simulink model "MarsEntry2"  (R2026a)
settings: Solver=ode45  StopTime=500  MaxStep=1  RelTol=1e-9  AbsTol=1e-10
settings Model: Creator=Ashwin  LastModifiedBy=aganesh
settings SFSimCC: SimGPUStackLimitPerThread=51200.0
settings RTWCC: GPUStackLimitPerThread=51200.0

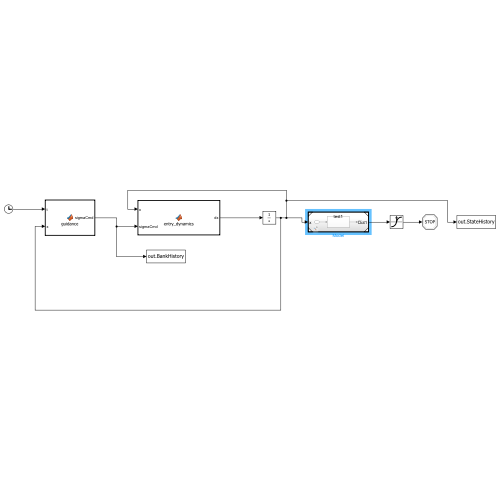
[thumbnail: Simulink's stored preview of the top-level diagram]
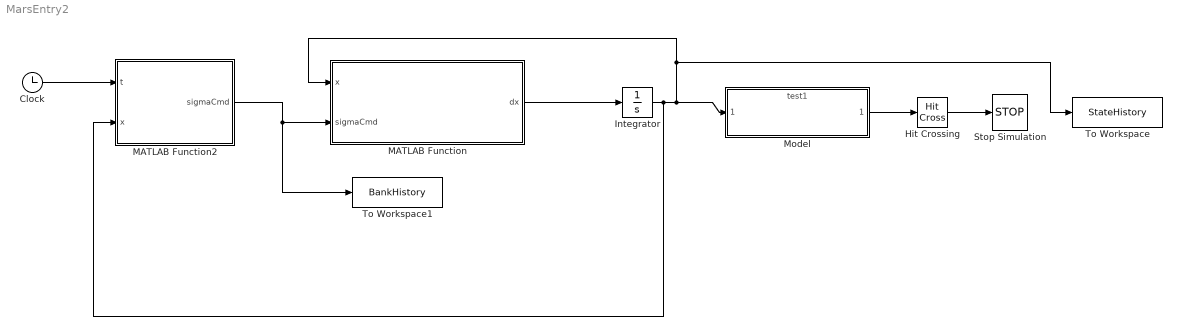
== system MarsEntry2 ==
  Clock : Clock
  Hit Crossing : HitCross  HitCrossingDirection=rising
  Integrator : Integrator  InitialCondition=[3397e3+125e3; -176.4*pi/180; -21.3*pi/180; 4700; -10*pi/180; -2.876*pi/180; 0]
  MATLAB Function : MATLAB Function  TreatAsAtomicUnit=on
  MATLAB Function2 : MATLAB Function  TreatAsAtomicUnit=on
  Model : ModelReference  ModelNameDialog=test1.slx  SimulationMode=Normal  ModelReferenceVersion=1.2
  Stop Simulation : Stop
  To Workspace : ToWorkspace  VariableName=StateHistory  SaveFormat=Timeseries  SampleTime=-1
  To Workspace1 : ToWorkspace  VariableName=BankHistory  SaveFormat=Timeseries  SampleTime=-1
  wires:
  MATLAB Function2/1(sigmaCmd) -> MATLAB Function/2(sigmaCmd), To Workspace1/1
  MATLAB Function/1(dx) -> Integrator/1
  Integrator/1 -> Model/1, MATLAB Function/1(x), To Workspace/1, MATLAB Function2/2(x)
  Clock/1 -> MATLAB Function2/1(t)
  Hit Crossing/1 -> Stop Simulation/1
  Model/1 -> Hit Crossing/1

== matlab function MarsEntry2/MATLAB Function2 ==
  settings: updateMethod=DISCRETE  sampleTime=1
  data: t input; sigmaCmd output; x input
function sigmaCmd = guidance(t,x)

coder.extrinsic('anpcg_update');
coder.extrinsic('anpcg_bank_direction');

persistent previousBank previousSign

if isempty(previousBank)
    previousBank = 100*pi/180;

    % Positive initial bank for this mission's heading error.
    previousSign = 1;
end

sigmaCmd = 0;

if t >= 175

    % Longitudinal guidance: determine bank magnitude
    nextBank = 0;
    nextBank = anpcg_update(x,previousBank);

    % Lateral guidance: determine bank direction
    nextSign = 1;
    nextSign = anpcg_bank_direction(x,nextBank,previousSign);

    previousBank = nextBank;
    previousSign = nextSign;

    sigmaCmd = nextSign*nextBank;
end

end

== matlab function MarsEntry2/MATLAB Function ==
  data: x input; dx output; sigmaCmd input
function dx = entry_dynamics(x, sigmaCmd)
% States: [r; theta; phi; V; gamma; psi; s]
% Distances in meters, time in seconds, angles in radians.

%% Mars constants
RMars = 3397e3;
mu    = 42828e9;
omega = 7.088e-5;

%% Human-mission vehicle
mass = 58800;
S    = 160;
CL   = 0.5236;
CD   = 0.9696;

beta = mass/(CD*S);
LD   = CL/CD;

%% Current states
r     = x(1);
phi   = x(3);
V     = x(4);
gamma = x(5);
psi   = x(6);

% Direct bank command: no actuator lag
sigma = sigmaCmd;

%% Atmosphere
h = r - RMars;

T = 1.4e-13*h^3 - 8.85e-9*h^2 ...
    - 1.245e-3*h + 205.36;

rho0 = 559.35/(188.95*T);
rho  = rho0*exp(-0.000105*h);

%% Gravity and aerodynamic accelerations
g = mu/r^2;
q = 0.5*rho*V^2;
D = q/beta;
L = LD*D;

%% Equations of motion
dx = zeros(7,1);

dx(1) = V*sin(gamma);

dx(2) = V*cos(gamma)*sin(psi)/(r*cos(phi));

dx(3) = V*cos(gamma)*cos(psi)/r;

dx(4) = -D - g*sin(gamma) ...
    + omega^2*r*cos(phi)*(sin(gamma)*cos(phi) ...
    - cos(gamma)*sin(phi)*cos(psi));

dx(5) = L*cos(sigma)/V ...
    + (V/r - g/V)*cos(gamma) ...
    + 2*omega*cos(phi)*sin(psi) ...
    + (omega^2*r/V)*cos(phi)*(cos(gamma)*cos(phi) ...
    + sin(gamma)*sin(phi)*cos(psi));

dx(6) = L*sin(sigma)/(V*cos(gamma)) ...
    + (V/r)*cos(gamma)*sin(psi)*tan(phi) ...
    + 2*omega*(sin(phi) - tan(gamma)*cos(phi)*cos(psi)) ...
    + (omega^2*r/(V*cos(gamma)))*sin(phi)*cos(phi)*sin(psi);

dx(7) = V*cos(gamma);

end
